simulink model "Model_with_Detector"  (R2024b)
settings: Solver=ode5  StartTime=0.0  StopTime=t_final  FixedStep=Ts  RelTol=1e-3
values from neighbouring files (symbols this model uses):
  A = (A + A')/2    [RKHS_fPCA.m]    (also in Run_file.m = [zeros(n_gen)                   eye(n_gen))
  Attack = randn()    [Run_file.m]
  B = [zeros(n_gen) zeros(n_gen, n_bus- n_gen) ... (first row only)    [Run_file.m]
  B_suscep = full(imag(Ybus))    [Run_file.m]
  C = [zeros(n_gen) eye(n_gen);          -L_ll\L_lg     zeros(n_bus-n_gen, n_gen)]    [Run_file.m]
  D = [zeros(n_gen)   zeros(n_gen,n_bus-n_gen); zeros(n_bus-n_gen,n_gen)   -L_ll^(-1)]    [Run_file.m]
  f = 1    [Run_file.m]
  G_conduct = full(real(Ybus))    [Run_file.m]
  gen_buses = mpc_agg.gen(:,1)    [Run_file.m]
  K_ctrl = place(A,B,P)    [Run_file.m]
  K_r = B_perp*A-K_ctrl    [Run_file.m]
  L = place(A.',C.',4*P).'    [Run_file.m]
  n_gen = size(gen,1)    [Run_file.m]
  n_x = size(A, 1)    [Run_file.m]
  n_y = size(C, 1)    [Run_file.m]
  T_detect_RKHS = (Window-1) * Ts    (= 0.19)    [Run_file.m]
  theta_m = bus(:,VA)*pi/180    [Run_file.m]
  Ts = 1e-2    (= 0.01)    [Run_file.m]
  Vm = bus(:,VM)    [Run_file.m]
  Window = 20    [Run_file.m]
  x_init = randn(n_x,1)    [Run_file.m]
  x_r = N_x*lambda    [Run_file.m]
undefined symbols (not defined in the file or in its folder): DiscIntNeverNeededParam
libraries: simulink x2
settings Model: Creator=Anubi  LastModifiedBy=rasla
settings ModelReferenceCC: EnableRefExpFcnMdlSchedulingChecks=on
settings RTWCC: GPUComputeCapability=3.5

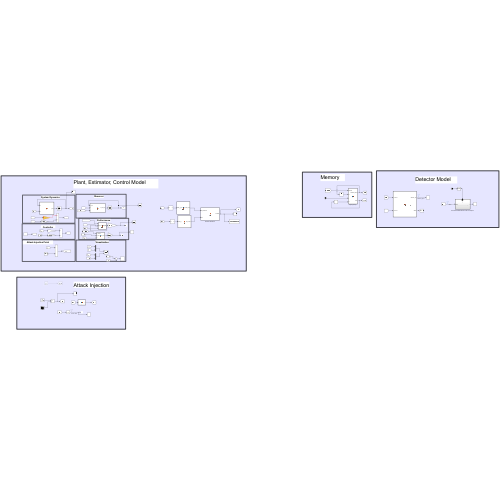
[thumbnail: Simulink's stored preview of the top-level diagram]
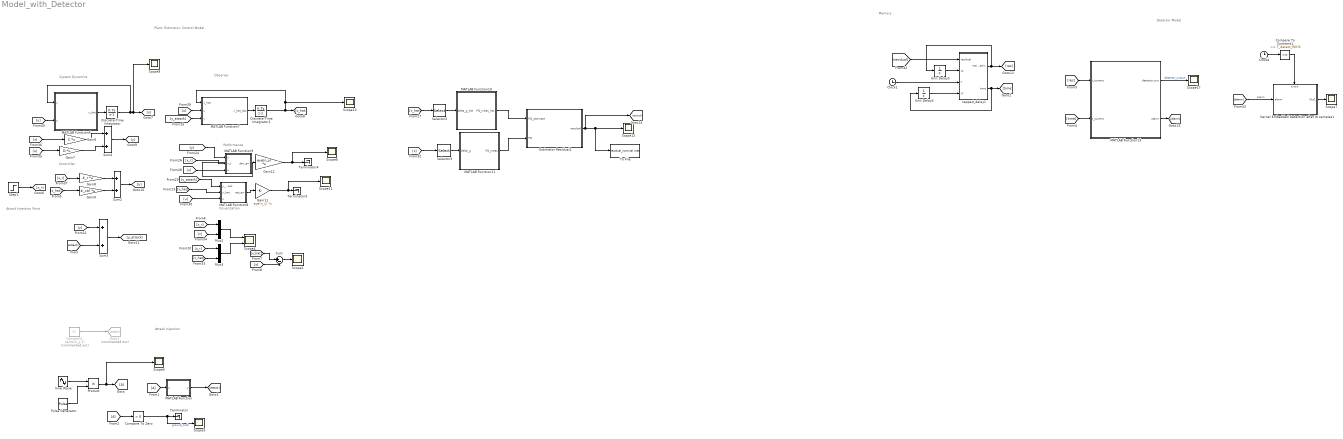
== system Model_with_Detector ==
  note: Attack Injection
  note: System Dynamics
  note: Controller
  note: Visualization
  note: Performance
  note: Attack Injection Point
  note: Plant, Estimator, Control Model
  note: Observer
  note: Memory
  note: Detector Model
  Clock1 : Clock
  Clock4 : Clock
  Compare To Constant1 : simulink/Logic and Bit Operations/Compare To Constant  relop=>=  const=T_detect_RKHS  OutDataTypeStr=boolean
  Compare To Zero : simulink/Logic and Bit Operations/Compare To Zero  relop=>  OutDataTypeStr=boolean
  Constant1 : Constant  Commented=on  Value=zeros(n_y,1)  SampleTime=Ts
  Discrete-Time Integrator : DiscreteIntegrator  InitialCondition=x_init  SampleTime=-1  ICPrevOutput=DiscIntNeverNeededParam  ICPrevScaledInput=DiscIntNeverNeededParam
  Discrete-Time Integrator1 : DiscreteIntegrator  InitialCondition=zeros(n_x,1)  SampleTime=-1  ICPrevOutput=DiscIntNeverNeededParam  ICPrevScaledInput=DiscIntNeverNeededParam
  Estimator Residual1 : MATLAB Function  TreatAsAtomicUnit=on
  From1 : From
  From2 : From
  Gain11 : Gain  Gain=eye(n_y)  Multiplication=Matrix(K*u) (u vector)
  Gain12 : Gain  Gain=eye(n_y)  Multiplication=Matrix(K*u) (u vector)
  Gain6 : Gain  Gain=C  Multiplication=Matrix(K*u) (u vector)
  Gain7 : Gain  Gain=D  Multiplication=Matrix(K*u) (u vector)
  Gain8 : Gain  Gain=-K_r  Multiplication=Matrix(K*u) (u vector)
  Gain9 : Gain  Gain=-K_ctrl  Multiplication=Matrix(K*u) (u vector)
  Goto : Goto
  Goto3 : Goto  Commented=on  GotoTag=attack
  Kernel Embedded Detection after W samples1 : Subsystem  TreatAsAtomicUnit=on
  MATLAB Function : MATLAB Function  TreatAsAtomicUnit=on
  MATLAB Function10 : MATLAB Function  TreatAsAtomicUnit=on
  MATLAB Function11 : MATLAB Function  TreatAsAtomicUnit=on
  MATLAB Function13 : MATLAB Function  TreatAsAtomicUnit=on
  MATLAB Function6 : MATLAB Function  TreatAsAtomicUnit=on
  MATLAB Function7 : MATLAB Function  TreatAsAtomicUnit=on
  MATLAB Function8 : MATLAB Function  TreatAsAtomicUnit=on
  MATLAB Function9 : MATLAB Function  TreatAsAtomicUnit=on
  Mux2 : Mux  Inputs=2
  Mux3 : Mux  Inputs=2
  Product : Product
  Pulse Generator : DiscretePulseGenerator  PulseType=Time based  Amplitude=Attack  Period=1/f  PulseWidth=50
  Scope{1,3,5..7,9..12,17} (10 alike) : Scope
  Scope4 : Scope  NumInputPorts=2
  Selector2 : Selector  InputPortWidth=n_x  IndexOptions=Index vector (dialog)  Indices=1:n_gen  OutputSizes=1
  Selector3 : Selector  InputPortWidth=n_x  IndexOptions=Index vector (dialog)  Indices=1:n_gen  OutputSizes=1
  Sine Wave : Sin  Amplitude=Attack  Frequency=2*pi*f  SampleTime=Ts
  Step1 : Step  Time=2  Before=zeros(n_x,1)  After=x_r  SampleTime=Ts
  Sum : Sum  Inputs=|+-
  Sum2 : Sum
  Sum3 : Sum
  Sum4 : Sum
  Terminator : Terminator
  Terminator3 : Terminator
  Terminator4 : Terminator
  To File : ToFile  Filename=residual_nominal.mat  MatrixName=residual_nominal  SaveFormat=Timeseries
  Unit Delay3 : UnitDelay  InitialCondition=zeros(Window,2*n_gen)  SampleTime=-1  HasFrameUpgradeWarning=on
  Unit Delay4 : UnitDelay  InitialCondition=zeros(Window,1)  SampleTime=-1  HasFrameUpgradeWarning=on
  tapped_delay1 : MATLAB Function  TreatAsAtomicUnit=on
  wires:
  Estimator Residual1/1(residual) -> [residual], To File/1, Scope12/1
  Sum3/1 -> [y_attack]
  Selector3/1 -> MATLAB Function11/1(delta_g)
  [u] -> MATLAB Function6/2(u)
  [u] -> MATLAB Function8/3(u)
  [x] -> Selector3/1
  [x_hat] -> Mux3/2
  Sum4/1 -> [y]
  Gain9/1 -> Sum2/2
  MATLAB Function9/1(dev_err) -> Gain12/1
  [y] -> Sum3/1
  Gain7/1 -> Sum4/2
  MATLAB Function8/1(est_err) -> Gain11/1
  MATLAB Function6/1(x_dot) -> Discrete-Time Integrator/1
  Selector2/1 -> MATLAB Function10/1(delta_g_hat)
  [y_attack] -> MATLAB Function8/1(y_attack)
  Gain6/1 -> Sum4/1
  Gain11/1 -> Scope11/1, Terminator3/1
  [u] -> MATLAB Function9/3(u)
  [x_hat] -> MATLAB Function8/2(x_hat)
  [x_r] -> MATLAB Function9/2(x_r)
  [u] -> MATLAB Function7/2(u)
  Discrete-Time Integrator1/1 -> Scope10/1, MATLAB Function7/1(x_hat), [x_hat]
  Sum2/1 -> [u]
  [y_attack] -> MATLAB Function7/3(y)
  [u] -> Gain7/1
  [x_r] -> Mux3/1
  [x_r] -> Gain8/1
  [x] -> Mux2/2
  [x_r] -> Mux2/1
  [x_hat] -> Selector2/1
  MATLAB Function7/1(x_hat_dot) -> Discrete-Time Integrator1/1
  Discrete-Time Integrator/1 -> Scope9/1, [x], MATLAB Function6/1(x)
  MATLAB Function11/1(PQ_meas) -> Estimator Residual1/2(PQ)
  [x_hat] -> Gain9/1
  Gain8/1 -> Sum2/1
  Gain12/1 -> Terminator4/1, Scope6/1
  Step1/1 -> [x_r]
  Mux2/1 -> Scope4/1
  [attack] -> Sum3/2
  Mux3/1 -> Scope4/2
  [x] -> Gain6/1
  MATLAB Function10/1(PQ_meas_hat) -> Estimator Residual1/1(PQ_estimate)
  [y] -> MATLAB Function9/1(y)
  Pulse Generator/1 -> Product/2
  Sine Wave/1 -> Product/1
  From1/1 -> MATLAB Function/1(u)
  Product/1 -> Scope5/1, Goto/1
  MATLAB Function/1(y) -> [attack]
  Compare To Zero/1 -> Scope3/1, Terminator/1  "ground_truth"
  From2/1 -> Compare To Zero/1
  Kernel Embedded Detection after W samples1/1(Out1) -> Scope7/1
  [time] -> MATLAB Function13/2(t_current)
  [residual] -> tapped_delay1/1(residual)
  Unit Delay3/1 -> tapped_delay1/2(ut)
  Unit Delay4/1 -> tapped_delay1/4(yt)
  tapped_delay1/2(time) -> Unit Delay4/1, [time]
  [res] -> MATLAB Function13/1(r_current)
  Clock1/1 -> tapped_delay1/3(t)
  Compare To Constant1/1 -> Kernel Embedded Detection after W samples1/Enable
  tapped_delay1/1(residual_matrix) -> Unit Delay3/1, [res]
  Clock4/1 -> Compare To Constant1/1
  [alarm] -> Kernel Embedded Detection after W samples1/1(alarm)  "alarm"
  MATLAB Function13/2(alarm) -> [alarm]
  MATLAB Function13/1(detector_out) -> Scope17/1  "detector_output"
  Constant1/1 -> Goto3/1
  [x_hat] -> Sum/1
  [x] -> Sum/2
  Sum/1 -> Scope1/1

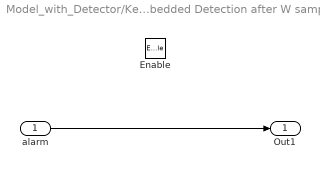
== system Model_with_Detector/Kernel Embedded Detection after W samples1 ==
  alarm : Inport
  Enable : EnablePort
  Out1 : Outport
  wires:
  alarm/1 -> Out1/1

== matlab function Model_with_Detector/MATLAB Function8 ==
  data: y_attack input; est_err output; x_hat input; C parameter; u input; D parameter
function est_err = fcn(y_attack,x_hat,C,u, D)

est_err = y_attack - (C*x_hat + D*u);

== matlab function Model_with_Detector/MATLAB Function9 ==
  data: y input; dev_err output; x_r input; C parameter; u input; D parameter
function dev_err = fcn(y,x_r,C,u, D)

dev_err = y - (C*x_r + D*u);

== matlab function Model_with_Detector/MATLAB Function13 ==
  data: detector_out output; r_current input; t_current input; params_detector parameter; alarm output
function [detector_out,alarm]  = kernel_embedded_detector(r_current, t_current,params_detector)
% Inputs:
%         r_current:        [matrix] stacked  current residuals 
%         t_current:        [vector] stacked current time 
%         params_detector:  [struct] parameter container

% Outputs: 
%          detector_out:   [scalar] detector energy 
%          alarm:          [binary] detector alarm

% Author: Abdrew Omiloli
% Date: June 15th, 2026

persistent idx alarm_buffer
%% Parameters
K_train          = params_detector.K_train;
Z_star           = params_detector.Z_star;
tau_KEFSD        = params_detector.tau_KEFSD;
tau_norm         = params_detector.tau_norm;
lambda           = params_detector.lambda;
sigma            = params_detector.sigma;           
t_train          = params_detector.time_extract;
Window           = params_detector.Window;
L                = 10;    % alarm window
m                = length(r_current(1,:)); % size of current residual 
Beta_star        = K_train \ Z_star;
kernel_fun       = @(t1,t2) exp(-(t1-t2).^2/(2*sigma^2)); % gausian kernel

if isempty(idx)
    idx = 0;
end
if isempty(alarm_buffer)
    alarm_buffer = false(1, L);
end
idx = min(idx+1,Window);
%% Instantaneous 2-norm residual based detector used before Window is full 
alarm_2_norm        = false;
norm_residual       = mean((r_current(end,:).^2));
if norm_residual > tau_norm
    alarm_2_norm = true;
end

%% Kernel based detection if window, W is full with samples
% Initializations
KEFSD_energy          = 0;
alarm_KEFSD           = false;
total_energy_store    = zeros(m,1);
proj_energy_store     = zeros(m,1);


if idx == Window
% Build Gram matrix (K_ww) for current window
K_ww = zeros(Window,Window);
for i=1:Window
    for j=1:Window
        K_ww(i,j) = kernel_fun(t_current(i), t_current(j));
    end
end

% Build cross-kernel matrix K_Wn (W x n)
K_Wn = zeros(Window,length(t_train));
for i=1:Window
    for j=1:length(t_train)
        K_Wn(i,j) = kernel_fun(t_current(i), t_train(j));
    end
end

% Compute measurement channel-wise energies 
 J_ch = zeros(m,1);
 for ch = 1:m
     r_ch    = r_current(:,ch);  % current residual channel wise 
     alpha_w = (K_ww + lambda*eye(Window)) \ r_ch; % kernel coefficient

     % RKHS norm of the estimated residual (g^hat)
     total_energy            = alpha_w' * K_ww * alpha_w;  
     total_energy_store(ch)  = total_energy;

     % Projected energy onto clean RKHS subspace
     proj_energy            = sum((alpha_w' * K_Wn * Beta_star).^2);
     proj_energy_store(ch)  = proj_energy;
    J_ch(ch)                = max(total_energy - proj_energy,0);
 end
     KEFSD_energy = mean(J_ch);
     if KEFSD_energy > tau_KEFSD
         alarm_KEFSD = true;
     end
end 

%% Switch detectors, before W, use residual based detector, when W is full
%  use KEFSD detector 
if idx < Window
 detector_out = norm_residual;
 alarm = alarm_2_norm;
 return;
end

detector_out = KEFSD_energy;
% alarm = alarm_func;


%% update sliding history of alarms
alarm_buffer = [alarm_buffer(:,2:end), alarm_KEFSD];
 
% output alarm based on majority vote decision
alarm = sum(alarm_buffer,2) >= ceil(0.6 * L);
end

== matlab function Model_with_Detector/tapped_delay1 ==
  data: residual input; residual_matrix output; ut input; t input; yt input; time output
function [residual_matrix,time] = fcn(residual,ut,t,yt)
%% tapped_delay_array
% shift columns from tapped matrix from bottom to top and appends most recent
ut(1:end-1,:) = ut(2:end,:);
ut(end,:) = residual(:)';
residual_matrix = ut;

yt(1:end-1,:) = yt(2:end,:);
yt(end,:) = t(:)';
time = yt;



% shift columns from tapped matrix to the left and appends most recent
% vector to the last column
%%% input
% ut(:,1:end-1) = ut(:,2:end);
% ut(:,end) = u;
% U = ut;
% %%% output
% yt(:,1:end-1) = yt(:,2:end);
% yt(:,end) = y;
% Y = yt;

== matlab function Model_with_Detector/MATLAB Function ==
  data: u input; y output; n_y parameter
function y = fcn(u,n_y)

y = repmat(u, [n_y,1]);

== matlab function Model_with_Detector/Estimator Residual1 ==
  data: PQ_estimate input; residual output; PQ input
function residual  = fcn(PQ_estimate, PQ)

residual = PQ_estimate - PQ;

== matlab function Model_with_Detector/MATLAB Function10 ==
  data: delta_g_hat input; PQ_meas_hat output; theta_m parameter; Vm parameter; G_conduct parameter; B_suscep parameter; gen_buses parameter; n_gen parameter
function PQ_meas_hat = fcn(delta_g_hat,theta_m,Vm,G_conduct, B_suscep, gen_buses, n_gen)

[Pe_g, Qe_g]         = electrical_power(delta_g_hat,G_conduct,B_suscep,n_gen,gen_buses,Vm,theta_m); 

PQ_meas_hat = [Pe_g; Qe_g];

== matlab function Model_with_Detector/MATLAB Function11 ==
  data: delta_g input; PQ_meas output; theta_m parameter; Vm parameter; G_conduct parameter; B_suscep parameter; gen_buses parameter; n_gen parameter
function PQ_meas = fcn(delta_g,theta_m,Vm,G_conduct, B_suscep, gen_buses, n_gen)

[Pe_g, Qe_g]         = electrical_power(delta_g,G_conduct,B_suscep,n_gen,gen_buses,Vm,theta_m); 

PQ_meas = [Pe_g; Qe_g];

== matlab function Model_with_Detector/MATLAB Function6 ==
  data: x input; x_dot output; u input; A parameter; B parameter
function x_dot = fcn(x,u,A, B)

x_dot = A*x + B*u;

== matlab function Model_with_Detector/MATLAB Function7 ==
  data: x_hat input; u input; x_hat_dot output; y input; A parameter; B parameter; C parameter; L parameter; D parameter
function x_hat_dot = fcn(x_hat,u,y,A, B, C,L, D)

x_hat_dot = A*x_hat + B*u + L*(y-C*x_hat) - L * D * u;
